simulink model "mecanum_control_benchmark"  (R2022b)
settings: Solver=FixedStepDiscrete  StartTime=0  StopTime=40  FixedStep=0.01  RelTol=1e-3
model workspace (MAT data in the model file):
  SLX_CASE_ID = 1
  SLX_CTRL = [10; 0.8; 2; 2; 0.5; 2; 2; 2.5; 5; 5; 4; 40; 40; 3.2; 1; 1; 0.15; 34; 34; 2.38; 3; 3; 2; 100; 100; 50; 0.01; 2; 0.2; 0.05; 0.3; 0.25]
  SLX_NU0 = [0; 0; 0]
  SLX_PLANT = [10; 0.8; 2; 2; 0.5; 0.05; 0.3; 0.25]
  SLX_Q0 = [2.2; -0.1; 1.74532925199]
  SLX_TRAJ_ID = 1
undefined symbols (not defined in the file or in its folder): DiscIntNeverNeededParam
settings Model: Creator=ADMIN  LastModifiedBy=ADMIN

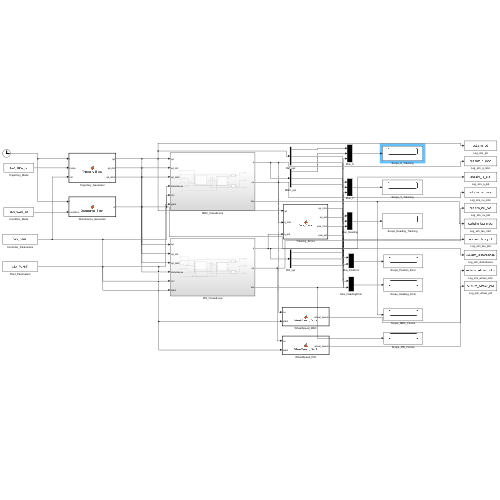
[thumbnail: Simulink's stored preview of the top-level diagram]
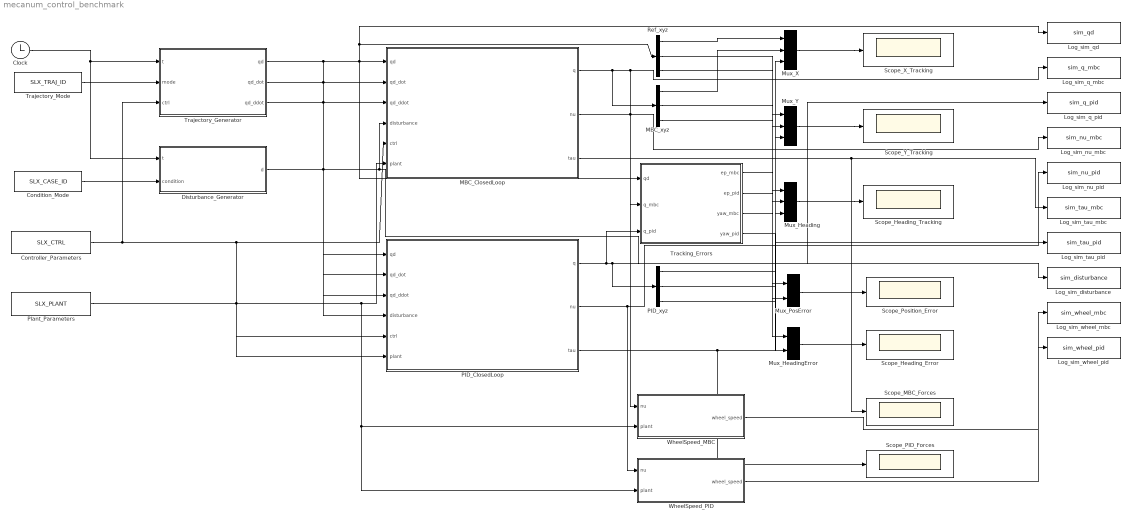
== system mecanum_control_benchmark ==
  Clock : Clock
  Condition_Mode : Constant  Value=SLX_CASE_ID
  Controller_Parameters : Constant  Value=SLX_CTRL
  Disturbance_Generator : MATLAB Function  TreatAsAtomicUnit=on
  Log_sim_disturbance : ToWorkspace  VariableName=sim_disturbance  SaveFormat=Timeseries  SampleTime=-1
  Log_sim_nu_mbc : ToWorkspace  VariableName=sim_nu_mbc  SaveFormat=Timeseries  SampleTime=-1
  Log_sim_nu_pid : ToWorkspace  VariableName=sim_nu_pid  SaveFormat=Timeseries  SampleTime=-1
  Log_sim_q_mbc : ToWorkspace  VariableName=sim_q_mbc  SaveFormat=Timeseries  SampleTime=-1
  Log_sim_q_pid : ToWorkspace  VariableName=sim_q_pid  SaveFormat=Timeseries  SampleTime=-1
  Log_sim_qd : ToWorkspace  VariableName=sim_qd  SaveFormat=Timeseries  SampleTime=-1
  Log_sim_tau_mbc : ToWorkspace  VariableName=sim_tau_mbc  SaveFormat=Timeseries  SampleTime=-1
  Log_sim_tau_pid : ToWorkspace  VariableName=sim_tau_pid  SaveFormat=Timeseries  SampleTime=-1
  Log_sim_wheel_mbc : ToWorkspace  VariableName=sim_wheel_mbc  SaveFormat=Timeseries  SampleTime=-1
  Log_sim_wheel_pid : ToWorkspace  VariableName=sim_wheel_pid  SaveFormat=Timeseries  SampleTime=-1
  MBC_ClosedLoop : Subsystem
  MBC_xyz : Demux  Outputs=3
  Mux_Heading : Mux  Inputs=3
  Mux_HeadingError : Mux  Inputs=2
  Mux_PosError : Mux  Inputs=2
  Mux_X : Mux  Inputs=3
  Mux_Y : Mux  Inputs=3
  PID_ClosedLoop : Subsystem
  PID_xyz : Demux  Outputs=3
  Plant_Parameters : Constant  Value=SLX_PLANT
  Ref_xyz : Demux  Outputs=3
  Scope_Heading_Error : Scope
  Scope_Heading_Tracking : Scope
  Scope_MBC_Forces : Scope
  Scope_PID_Forces : Scope
  Scope_Position_Error : Scope
  Scope_X_Tracking : Scope
  Scope_Y_Tracking : Scope
  Tracking_Errors : MATLAB Function  TreatAsAtomicUnit=on
  Trajectory_Generator : MATLAB Function  TreatAsAtomicUnit=on
  Trajectory_Mode : Constant  Value=SLX_TRAJ_ID
  WheelSpeed_MBC : MATLAB Function  TreatAsAtomicUnit=on
  WheelSpeed_PID : MATLAB Function  TreatAsAtomicUnit=on
  wires:
  Clock/1 -> Trajectory_Generator/1(t), Disturbance_Generator/1(t)
  Trajectory_Mode/1 -> Trajectory_Generator/2(mode)
  Controller_Parameters/1 -> MBC_ClosedLoop/5(ctrl), PID_ClosedLoop/5(ctrl), Trajectory_Generator/3(ctrl)
  Condition_Mode/1 -> Disturbance_Generator/2(condition)
  Trajectory_Generator/1(qd) -> MBC_ClosedLoop/1(qd), Ref_xyz/1, Log_sim_qd/1, Tracking_Errors/1(qd), PID_ClosedLoop/1(qd)
  Trajectory_Generator/2(qd_dot) -> MBC_ClosedLoop/2(qd_dot), PID_ClosedLoop/2(qd_dot)
  Trajectory_Generator/3(qd_ddot) -> MBC_ClosedLoop/3(qd_ddot), PID_ClosedLoop/3(qd_ddot)
  Disturbance_Generator/1(d) -> MBC_ClosedLoop/4(disturbance), Log_sim_disturbance/1, PID_ClosedLoop/4(disturbance)
  Plant_Parameters/1 -> WheelSpeed_MBC/2(plant), WheelSpeed_PID/2(plant), MBC_ClosedLoop/6(plant), PID_ClosedLoop/6(plant)
  MBC_ClosedLoop/1(q) -> Tracking_Errors/2(q_mbc), Log_sim_q_mbc/1, MBC_xyz/1
  PID_ClosedLoop/1(q) -> PID_xyz/1, Log_sim_q_pid/1, Tracking_Errors/3(q_pid)
  Ref_xyz/1 -> Mux_X/1
  MBC_xyz/1 -> Mux_X/2
  PID_xyz/1 -> Mux_X/3
  Mux_X/1 -> Scope_X_Tracking/1
  Ref_xyz/2 -> Mux_Y/1
  MBC_xyz/2 -> Mux_Y/2
  PID_xyz/2 -> Mux_Y/3
  Mux_Y/1 -> Scope_Y_Tracking/1
  Ref_xyz/3 -> Mux_Heading/1
  MBC_xyz/3 -> Mux_Heading/2
  PID_xyz/3 -> Mux_Heading/3
  Mux_Heading/1 -> Scope_Heading_Tracking/1
  Tracking_Errors/1(ep_mbc) -> Mux_PosError/1
  Tracking_Errors/2(ep_pid) -> Mux_PosError/2
  Mux_PosError/1 -> Scope_Position_Error/1
  Tracking_Errors/3(yaw_mbc) -> Mux_HeadingError/1
  Tracking_Errors/4(yaw_pid) -> Mux_HeadingError/2
  Mux_HeadingError/1 -> Scope_Heading_Error/1
  MBC_ClosedLoop/3(tau) -> Scope_MBC_Forces/1, Log_sim_tau_mbc/1
  PID_ClosedLoop/3(tau) -> Scope_PID_Forces/1, Log_sim_tau_pid/1
  MBC_ClosedLoop/2(nu) -> WheelSpeed_MBC/1(nu), Log_sim_nu_mbc/1
  PID_ClosedLoop/2(nu) -> WheelSpeed_PID/1(nu), Log_sim_nu_pid/1
  WheelSpeed_MBC/1(wheel_speed) -> Log_sim_wheel_mbc/1
  WheelSpeed_PID/1(wheel_speed) -> Log_sim_wheel_pid/1

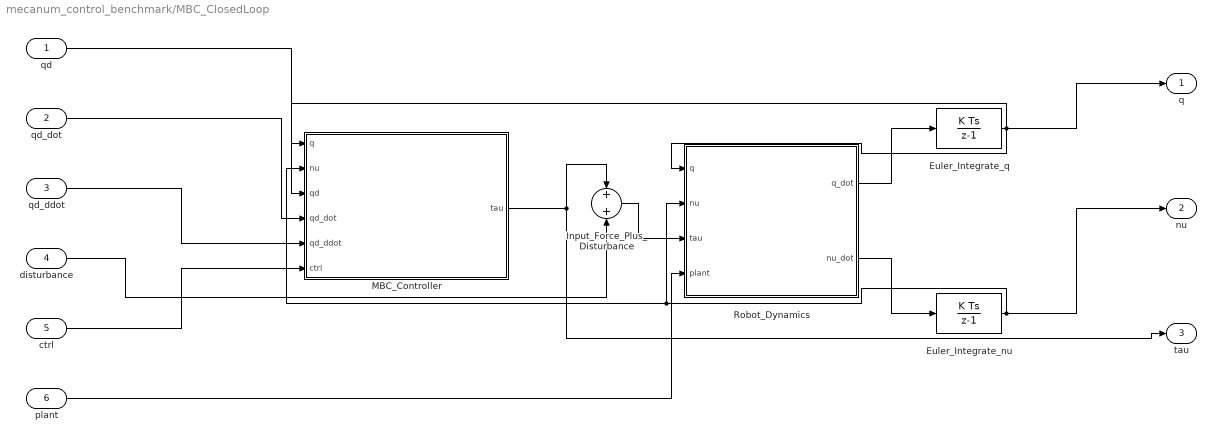
== system mecanum_control_benchmark/MBC_ClosedLoop ==
  qd : Inport
  qd_dot : Inport  Port=2
  qd_ddot : Inport  Port=3
  disturbance : Inport  Port=4
  ctrl : Inport  Port=5
  plant : Inport  Port=6
  Euler_Integrate_nu : DiscreteIntegrator  InitialCondition=SLX_NU0  SampleTime=0.01  ICPrevOutput=DiscIntNeverNeededParam  ICPrevScaledInput=DiscIntNeverNeededParam
  Euler_Integrate_q : DiscreteIntegrator  InitialCondition=SLX_Q0  SampleTime=0.01  ICPrevOutput=DiscIntNeverNeededParam  ICPrevScaledInput=DiscIntNeverNeededParam
  Input_Force_Plus_Disturbance : Sum
  MBC_Controller : MATLAB Function  TreatAsAtomicUnit=on
  Robot_Dynamics : MATLAB Function  TreatAsAtomicUnit=on
  q : Outport
  nu : Outport  Port=2
  tau : Outport  Port=3
  wires:
  qd_ddot/1 -> MBC_Controller/5(qd_ddot)
  ctrl/1 -> MBC_Controller/6(ctrl)
  qd/1 -> MBC_Controller/3(qd)
  qd_dot/1 -> MBC_Controller/4(qd_dot)
  MBC_Controller/1(tau) -> Input_Force_Plus_Disturbance/1, tau/1
  disturbance/1 -> Input_Force_Plus_Disturbance/2
  Input_Force_Plus_Disturbance/1 -> Robot_Dynamics/3(tau)
  plant/1 -> Robot_Dynamics/4(plant)
  Robot_Dynamics/1(q_dot) -> Euler_Integrate_q/1
  Robot_Dynamics/2(nu_dot) -> Euler_Integrate_nu/1
  Euler_Integrate_q/1 -> MBC_Controller/1(q), Robot_Dynamics/1(q), q/1
  Euler_Integrate_nu/1 -> MBC_Controller/2(nu), Robot_Dynamics/2(nu), nu/1

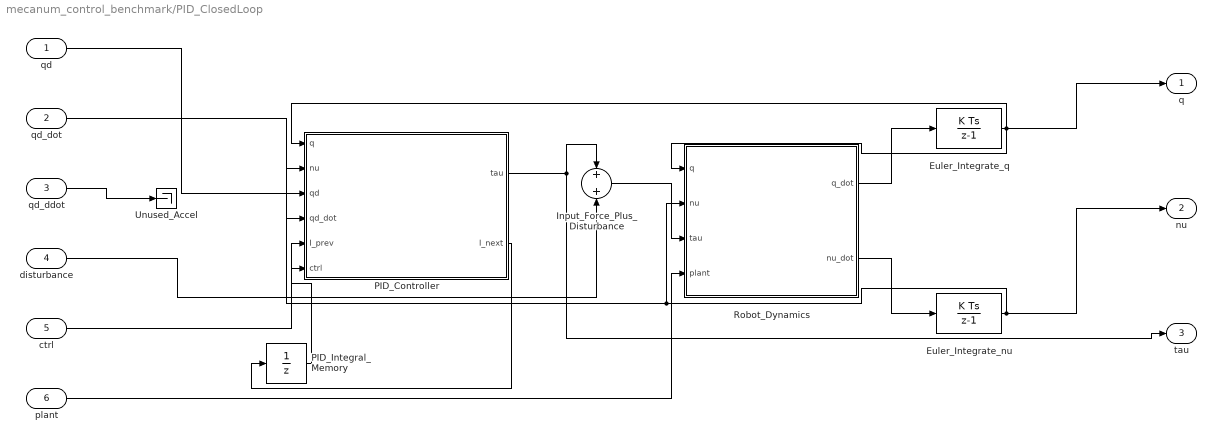
== system mecanum_control_benchmark/PID_ClosedLoop ==
  qd : Inport
  qd_dot : Inport  Port=2
  qd_ddot : Inport  Port=3
  disturbance : Inport  Port=4
  ctrl : Inport  Port=5
  plant : Inport  Port=6
  Euler_Integrate_nu : DiscreteIntegrator  InitialCondition=SLX_NU0  SampleTime=0.01  ICPrevOutput=DiscIntNeverNeededParam  ICPrevScaledInput=DiscIntNeverNeededParam
  Euler_Integrate_q : DiscreteIntegrator  InitialCondition=SLX_Q0  SampleTime=0.01  ICPrevOutput=DiscIntNeverNeededParam  ICPrevScaledInput=DiscIntNeverNeededParam
  Input_Force_Plus_Disturbance : Sum
  PID_Controller : MATLAB Function  TreatAsAtomicUnit=on
  PID_Integral_Memory : UnitDelay  InitialCondition=[0;0;0]  SampleTime=0.01  HasFrameUpgradeWarning=on
  Robot_Dynamics : MATLAB Function  TreatAsAtomicUnit=on
  Unused_Accel : Terminator
  q : Outport
  nu : Outport  Port=2
  tau : Outport  Port=3
  wires:
  PID_Integral_Memory/1 -> PID_Controller/5(I_prev)
  PID_Controller/2(I_next) -> PID_Integral_Memory/1
  ctrl/1 -> PID_Controller/6(ctrl)
  qd_ddot/1 -> Unused_Accel/1
  qd/1 -> PID_Controller/3(qd)
  qd_dot/1 -> PID_Controller/4(qd_dot)
  PID_Controller/1(tau) -> Input_Force_Plus_Disturbance/1, tau/1
  disturbance/1 -> Input_Force_Plus_Disturbance/2
  Input_Force_Plus_Disturbance/1 -> Robot_Dynamics/3(tau)
  plant/1 -> Robot_Dynamics/4(plant)
  Robot_Dynamics/1(q_dot) -> Euler_Integrate_q/1
  Robot_Dynamics/2(nu_dot) -> Euler_Integrate_nu/1
  Euler_Integrate_q/1 -> PID_Controller/1(q), Robot_Dynamics/1(q), q/1
  Euler_Integrate_nu/1 -> PID_Controller/2(nu), Robot_Dynamics/2(nu), nu/1

== matlab function mecanum_control_benchmark/Disturbance_Generator ==
  data: t input; d output; condition input
function d = Disturbance_Block(t,condition)
% condition=1 nominal, 2 payload, 3 disturbance.
d = zeros(3,1);
if (condition == 3) && (t >= 15) && (t <= 20)
    d = [15;-10;2];
end
end

== matlab function mecanum_control_benchmark/Trajectory_Generator ==
  data: t input; qd output; mode input; ctrl input; qd_dot output; qd_ddot output
function [qd,qd_dot,qd_ddot] = Trajectory_Block(t, mode, ctrl)
% 1=circle, 2=ellipse, 3=figure-eight, 4=lateral sine.
% Exact analytic formulas from the extended MATLAB benchmark.
w = ctrl(29);
Rtraj = ctrl(28);
if mode == 1
    x = Rtraj*cos(w*t); y = Rtraj*sin(w*t);
    vx = -Rtraj*w*sin(w*t); vy = Rtraj*w*cos(w*t);
    ax = -Rtraj*w*w*cos(w*t); ay = -Rtraj*w*w*sin(w*t);
    theta = w*t + pi/2; omega = w; alpha = 0;
elseif mode == 2
    a = 2; b = 1.2;
    x = a*cos(w*t); y = b*sin(w*t);
    vx = -a*w*sin(w*t); vy = b*w*cos(w*t);
    ax = -a*w*w*cos(w*t); ay = -b*w*w*sin(w*t);
    jx = a*w*w*w*sin(w*t); jy = -b*w*w*w*cos(w*t);
    [theta,omega,alpha] = tangent_motion(vx,vy,ax,ay,jx,jy);
elseif mode == 3
    a = 2; b = 1.4;
    x = a*sin(w*t); y = 0.5*b*sin(2*w*t);
    vx = a*w*cos(w*t); vy = b*w*cos(2*w*t);
    ax = -a*w*w*sin(w*t); ay = -2*b*w*w*sin(2*w*t);
    jx = -a*w*w*w*cos(w*t); jy = -4*b*w*w*w*cos(2*w*t);
    [theta,omega,alpha] = tangent_motion(vx,vy,ax,ay,jx,jy);
else
    v = 0.35; A = 0.6; ws = 0.4;
    x = v*t; y = A*sin(ws*t);
    vx = v; vy = A*ws*cos(ws*t);
    ax = 0; ay = -A*ws*ws*sin(ws*t);
    theta = 0; omega = 0; alpha = 0;
end
qd = [x;y;theta];
qd_dot = [vx;vy;omega];
qd_ddot = [ax;ay;alpha];
end

function [theta,omega,alpha] = tangent_motion(vx,vy,ax,ay,jx,jy)
s2 = vx*vx + vy*vy;
crossVA = vx*ay - vy*ax;
theta = atan2(vy,vx);
omega = crossVA/s2;
alpha = (vx*jy - vy*jx)/s2 - 2*crossVA*(vx*ax + vy*ay)/(s2*s2);
end

== matlab function mecanum_control_benchmark/MBC_ClosedLoop/MBC_Controller ==
  data: q input; tau output; nu input; qd input; qd_dot input; qd_ddot input; ctrl input
function tau = MBC_Block(q,nu,qd,qd_dot,qd_ddot,ctrl)
% Exact equivalent of uploaded controller_MBC.m (simplified MBC).
% ctrl indices documented in README; output [Fx;Fy;Mz] in BODY frame.
theta = q(3);
error = qd-q;
error(3) = atan2(sin(error(3)),cos(error(3)));
R = [cos(theta),-sin(theta),0;sin(theta),cos(theta),0;0,0,1];
Kp = diag(ctrl(6:8));
Kv = diag(ctrl(9:11));
qdot_ref = qd_dot + Kp*error;
nu_d = R'*qdot_ref;
nu_ddot_ff = R'*qd_ddot;
e_v = nu_d-nu;
nu_dot_cmd = nu_ddot_ff + Kv*e_v;
m = ctrl(1); Iz = ctrl(2);
M = diag([m;m;Iz]); D = diag(ctrl(3:5));
w = nu(3);
C = [0,-m*w,0;m*w,0,0;0,0,0];
tau = M*nu_dot_cmd + C*nu + D*nu;
tau = max(min(tau,ctrl(24:26)),-ctrl(24:26));
end

== matlab function mecanum_control_benchmark/MBC_ClosedLoop/Robot_Dynamics ==
  data: q input; q_dot output; nu input; tau input; plant input; nu_dot output
function [q_dot,nu_dot] = Plant_Block(q,nu,tau,plant)
% Exactly mirrors robot_dynamics.m. No wheel slip or motor model.
theta = q(3);
R = [cos(theta),-sin(theta),0;sin(theta),cos(theta),0;0,0,1];
q_dot = R*nu;
m = plant(1); Iz = plant(2);
M = diag([m;m;Iz]);
D = diag(plant(3:5));
w = nu(3);
C = [0,-m*w,0;m*w,0,0;0,0,0];
nu_dot = M \ (tau - C*nu - D*nu);
end

== matlab function mecanum_control_benchmark/PID_ClosedLoop/PID_Controller ==
  data: q input; tau output; nu input; qd input; qd_dot input; I_prev input; ctrl input; I_next output
function [tau,I_next] = PID_Block(q,nu,qd,qd_dot,I_prev,ctrl)
% Exact equivalent of controller_PID.m including integral before output.
theta = q(3);
R = [cos(theta),-sin(theta),0;sin(theta),cos(theta),0;0,0,1];
q_dot = R*nu;
error = qd-q;
error(3) = atan2(sin(error(3)),cos(error(3)));
error_dot = qd_dot-q_dot;
I_next = I_prev + error*ctrl(27);
I_next = max(min(I_next,ctrl(21:23)),-ctrl(21:23));
Kp = diag(ctrl(12:14));
Ki = diag(ctrl(15:17));
Kd = diag(ctrl(18:20));
tau_world = Kp*error + Ki*I_next + Kd*error_dot;
tau = R'*tau_world;
tau = max(min(tau,ctrl(24:26)),-ctrl(24:26));
end

== matlab function mecanum_control_benchmark/PID_ClosedLoop/Robot_Dynamics ==
  data: q input; q_dot output; nu input; tau input; plant input; nu_dot output
function [q_dot,nu_dot] = Plant_Block(q,nu,tau,plant)
% Exactly mirrors robot_dynamics.m. No wheel slip or motor model.
theta = q(3);
R = [cos(theta),-sin(theta),0;sin(theta),cos(theta),0;0,0,1];
q_dot = R*nu;
m = plant(1); Iz = plant(2);
M = diag([m;m;Iz]);
D = diag(plant(3:5));
w = nu(3);
C = [0,-m*w,0;m*w,0,0;0,0,0];
nu_dot = M \ (tau - C*nu - D*nu);
end

== matlab function mecanum_control_benchmark/Tracking_Errors ==
  data: qd input; ep_mbc output; q_mbc input; q_pid input; ep_pid output; yaw_mbc output; yaw_pid output
function [ep_mbc,ep_pid,yaw_mbc,yaw_pid] = Error_Block(qd,q_mbc,q_pid)
e_mbc = qd - q_mbc;
e_pid = qd - q_pid;
e_mbc(3) = atan2(sin(e_mbc(3)),cos(e_mbc(3)));
e_pid(3) = atan2(sin(e_pid(3)),cos(e_pid(3)));
ep_mbc = hypot(e_mbc(1),e_mbc(2));
ep_pid = hypot(e_pid(1),e_pid(2));
yaw_mbc = e_mbc(3);
yaw_pid = e_pid(3);
end

== matlab function mecanum_control_benchmark/WheelSpeed_MBC ==
  data: nu input; wheel_speed output; plant input
function wheel_speed = WheelSpeed_Block(nu,plant)
% Diagnostic only: 4 wheel rates rad/s, no actuator saturation.
r = plant(6); a = plant(7) + plant(8);
Jm = (1/r)*[1,-1,-a;1,1,a;1,1,-a;1,-1,a];
wheel_speed = Jm*nu;
end

== matlab function mecanum_control_benchmark/WheelSpeed_PID ==
  data: nu input; wheel_speed output; plant input
function wheel_speed = WheelSpeed_Block(nu,plant)
% Diagnostic only: 4 wheel rates rad/s, no actuator saturation.
r = plant(6); a = plant(7) + plant(8);
Jm = (1/r)*[1,-1,-a;1,1,a;1,1,-a;1,-1,a];
wheel_speed = Jm*nu;
end
